simulink model "simulink7_lqr_balance_control"  (R2026b)
settings: Solver=ode113  StopTime=20.0  FixedStep=0.0001
values from neighbouring files (symbols this model uses):
  A = [0 0 1 0 ... (first row only)    [QUBE2_ROTPEN_ABCD_eqns.m]
  B = kt * B / Rm    [QUBE2_ROTPEN_ABCD_eqns.m]
  C = eye(4,4)    [QUBE2_ROTPEN_ABCD_eqns.m]
  cons = cons_deg*(pi/180)    (= 0.523598775598)    [setup_qube2_rotpen.m]
  D = zeros(4,1)    [QUBE2_ROTPEN_ABCD_eqns.m]
  K = lqr(A, B, Q, R)    [setup_qube2_rotpen.m]
  Kbis = lqr(A, B, Qbis, R)    [setup_qube2_rotpen.m]
  kr = [1; 0; 0; 0]    [setup_qube2_rotpen.m]
  Kter = lqr(A, B, Qter, R)    [setup_qube2_rotpen.m]
  x0 = [0; 0; 0; 0]    [setup_qube2_rotpen.m]
settings Model: Creator=leelou  LastModifiedBy=leelou

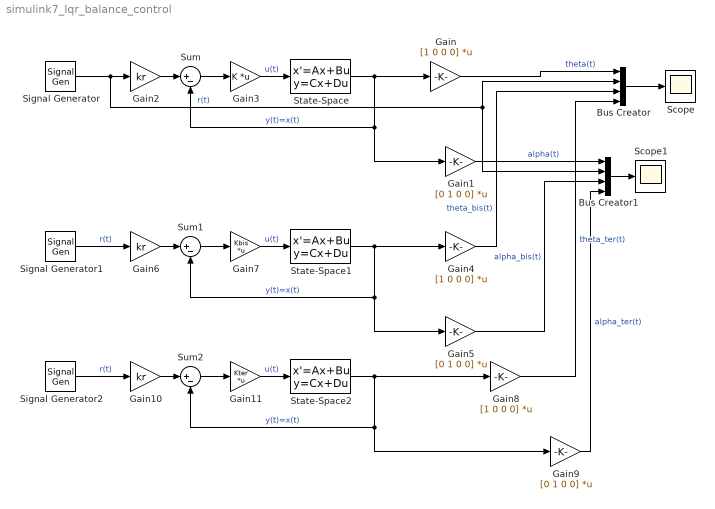
== system simulink7_lqr_balance_control ==
  Bus Creator : BusCreator  Inputs=4
  Bus Creator1 : BusCreator  Inputs=4
  Gain : Gain  Gain=[1 0 0 0]  Multiplication=Matrix(K*u) (u vector)
  Gain1 : Gain  Gain=[0 1 0 0]  Multiplication=Matrix(K*u) (u vector)
  Gain10 : Gain  Gain=kr
  Gain11 : Gain  Gain=Kter  Multiplication=Matrix(K*u) (u vector)
  Gain2 : Gain  Gain=kr
  Gain3 : Gain  Gain=K  Multiplication=Matrix(K*u) (u vector)
  Gain4 : Gain  Gain=[1 0 0 0]  Multiplication=Matrix(K*u) (u vector)
  Gain5 : Gain  Gain=[0 1 0 0]  Multiplication=Matrix(K*u) (u vector)
  Gain6 : Gain  Gain=kr
  Gain7 : Gain  Gain=Kbis  Multiplication=Matrix(K*u) (u vector)
  Gain8 : Gain  Gain=[1 0 0 0]  Multiplication=Matrix(K*u) (u vector)
  Gain9 : Gain  Gain=[0 1 0 0]  Multiplication=Matrix(K*u) (u vector)
  Scope : Scope
      settings: ActiveDisplayYMinimum=-0.71360457864400817  ActiveDisplayYMaximum=0.71357943438097571
  Scope1 : Scope
      settings: ActiveDisplayYMinimum=-0.65449846949787349  ActiveDisplayYMaximum=0.65449846949787349
  Signal Generator : SignalGenerator  WaveForm=square  Amplitude=cons  Frequency=0.125
  Signal Generator1 : SignalGenerator  WaveForm=square  Amplitude=cons  Frequency=0.125
  Signal Generator2 : SignalGenerator  WaveForm=square  Amplitude=cons  Frequency=0.125
  State-Space : StateSpace  A=A  B=B  C=C  D=D  InitialCondition=x0
  State-Space1 : StateSpace  A=A  B=B  C=C  D=D  InitialCondition=x0
  State-Space2 : StateSpace  A=A  B=B  C=C  D=D  InitialCondition=x0
  Sum : Sum  Inputs=|+-
  Sum1 : Sum  Inputs=|+-
  Sum2 : Sum  Inputs=|+-
  wires:
  Bus Creator/1 -> Scope/1
  Bus Creator1/1 -> Scope1/1
  Gain1/1 -> Bus Creator1/1  "alpha(t)"
  State-Space/1 -> Gain1/1, Sum/2, Gain/1  "y(t)=x(t)"
  Gain2/1 -> Sum/1
  Gain3/1 -> State-Space/1  "u(t)"
  Sum/1 -> Gain3/1
  Signal Generator/1 -> Bus Creator/2, Bus Creator1/2, Gain2/1  "r(t)"
  Gain/1 -> Bus Creator/1  "theta(t)"
  Gain4/1 -> Bus Creator/3  "theta_bis(t)"
  Gain5/1 -> Bus Creator1/3  "alpha_bis(t)"
  Sum1/1 -> Gain7/1
  Gain7/1 -> State-Space1/1  "u(t)"
  Signal Generator1/1 -> Gain6/1  "r(t)"
  Gain6/1 -> Sum1/1
  State-Space1/1 -> Gain5/1, Sum1/2, Gain4/1  "y(t)=x(t)"
  Gain10/1 -> Sum2/1
  State-Space2/1 -> Gain9/1, Sum2/2, Gain8/1  "y(t)=x(t)"
  Sum2/1 -> Gain11/1
  Gain11/1 -> State-Space2/1  "u(t)"
  Signal Generator2/1 -> Gain10/1  "r(t)"
  Gain8/1 -> Bus Creator/4  "theta_ter(t)"
  Gain9/1 -> Bus Creator1/4  "alpha_ter(t)"
